simulink model "MotorDC_Simscape"  (R2026a)
settings: Solver=ode23t  StopTime=5
values from neighbouring files (symbols this model uses):
  b = 0.0012    [crear_motor_simscape.m]    (also in crear_motor_simulink.m; mat.m)
  Kt = 0.01    [crear_motor_simscape.m]    (also in crear_motor_simulink.m; mat.m)
  Ra = 2    [crear_motor_simscape.m]    (also in crear_motor_simulink.m; mat.m)
libraries: fl_lib x10, nesl_utility x4
settings Model: Creator=jmlc2  LastModifiedBy=jmlc2

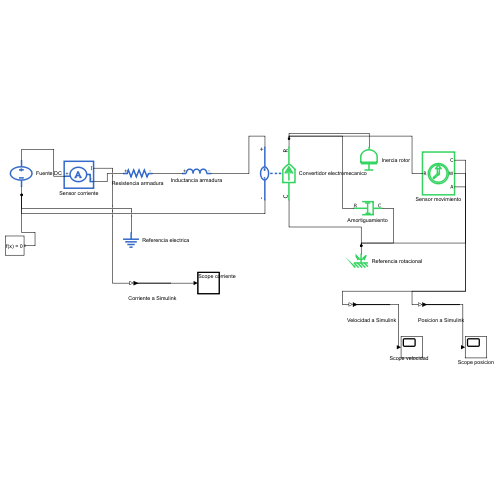
[thumbnail: Simulink's stored preview of the top-level diagram]
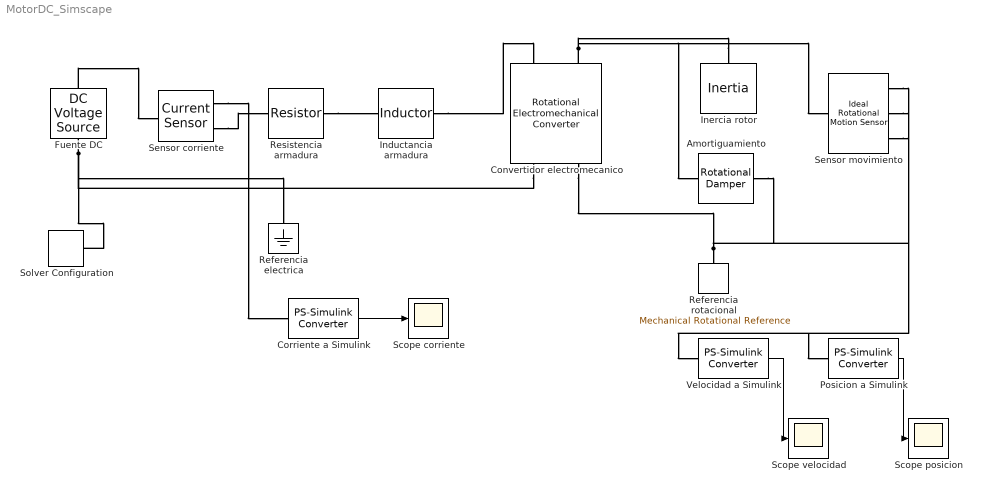
== system MotorDC_Simscape ==
  Amortiguamiento : fl_lib/Mechanical/Rotational Elements/Rotational Damper  D=b N*m*s/rad  w_specify=off  w_priority=None  w=0 rad/s  w_nominal_specify=off  w_nominal_value=1  w_nominal_unit=rad/s  t_specify=off  t_priority=None  t=0 N*m  t_nominal_specify=off  t_nominal_value=1  t_nominal_unit=N*m
  Convertidor electromecanico : fl_lib/Electrical/Electrical Elements/Rotational Electromechanical Converter  K=Kt V*s/rad  i_specify=off  i_priority=None  i=0 A  i_nominal_specify=off  i_nominal_value=1  i_nominal_unit=A  v_specify=off  v_priority=None  v=0 V  v_nominal_specify=off  v_nominal_value=1  v_nominal_unit=V  t_specify=off  t_priority=None  t=0 N*m  t_nominal_specify=off  t_nominal_value=1  t_nominal_unit=N*m  w_specify=off  w_priority=None  w=0 rad/s  w_nominal_specify=off  w_nominal_value=1  w_nominal_unit=rad/s
  Corriente a Simulink : nesl_utility/PS-Simulink Converter  PhysicalDomain=network_engine_domain  SubClassName=ps_output  LeftPortType=input  RightPortType=output  PseudoPeriodic=off  Frequencies=[]  VectorFormat=inherit  Unit=A  AffineConversion=off
  Fuente DC : fl_lib/Electrical/Electrical Sources/DC Voltage Source  v0=va V
  Inductancia armadura : fl_lib/Electrical/Electrical Elements/Inductor  l=La H  r=0 Ohm  g=1e-9 1/Ohm  i_specify=off  i_priority=None  i=0 A  i_nominal_specify=off  i_nominal_value=1  i_nominal_unit=A  v_specify=off  v_priority=None  v=0 V  v_nominal_specify=off  v_nominal_value=1  v_nominal_unit=V  i_L_specify=off  i_L_priority=High  i_L=0 A  i_L_nominal_specify=off  i_L_nominal_value=1  i_L_nominal_unit=A
  Inercia rotor : fl_lib/Mechanical/Rotational Elements/Inertia  inertia=J kg*m^2  num_ports=foundation.enum.numPorts2.one  w_specify=off  w_priority=High  w=0 rad/s  w_nominal_specify=off  w_nominal_value=1  w_nominal_unit=rad/s  t_specify=off  t_priority=None  t=0 N*m  t_nominal_specify=off  t_nominal_value=1  t_nominal_unit=N*m
  Posicion a Simulink : nesl_utility/PS-Simulink Converter  PhysicalDomain=network_engine_domain  SubClassName=ps_output  LeftPortType=input  RightPortType=output  PseudoPeriodic=off  Frequencies=[]  VectorFormat=inherit  Unit=rad  AffineConversion=off
  Referencia electrica : fl_lib/Electrical/Electrical Elements/Electrical Reference
  Referencia rotacional : fl_lib/Mechanical/Rotational Elements/Mechanical Rotational Reference
  Resistencia armadura : fl_lib/Electrical/Electrical Elements/Resistor  R=Ra Ohm  i_specify=off  i_priority=None  i=0 A  i_nominal_specify=off  i_nominal_value=1  i_nominal_unit=A  v_specify=off  v_priority=None  v=0 V  v_nominal_specify=off  v_nominal_value=1  v_nominal_unit=V
  Scope corriente : Scope
      settings: TimeSpan=5  ActiveDisplayYMinimum=0  ActiveDisplayYMaximum=6
  Scope posicion : Scope
      settings: TimeSpan=5  ActiveDisplayYMinimum=0  ActiveDisplayYMaximum=250
  Scope velocidad : Scope
      settings: TimeSpan=5  ActiveDisplayYMinimum=0  ActiveDisplayYMaximum=50
  Sensor corriente : fl_lib/Electrical/Electrical Sensors/Current Sensor
  Sensor movimiento : fl_lib/Mechanical/Mechanical Sensors/Ideal Rotational Motion Sensor  reference=foundation.enum.MeasurementReference.difference  acceleration_port=false  velocity_port=true  position_port=true  wrap_angle=false  offset=0 rad
  Solver Configuration : nesl_utility/Solver Configuration  PhysicalDomain=network_engine_domain  SubClassName=solver  LeftPortType=input  RightPortType=generic  Tones=[]  Harmonics=[]  SimulateNoise=off  Profile=off  UseLocalSampling=off  EnableSwitchedLinearOptims=on  FrequencyDomain=off  UseCCode=off  RelTol=0.001  AbsTol=0.001  MinStep=1e-09  ToWorkspace=off  RevertToSquareIcSolve=off  NumHomotopyIterations=100  PhasorMode=off  PhasorModeNumHarmonics=1  ConsistencySolver=NEWTON_XTOL_AFTER_FTOL  CanonicalOrdering=CANONICAL  OptimizeIntermediates=OPTIMIZED  IndexReductionMethod=DerivativeReplacement  DoDC=off  ResidualTolerance=1e-09  ConsistencyTolSource=GLOBAL  ConsistencyAbsTol=0.001  ConsistencyRelTol=0.001  ConsistencyTolFactor=0.001  UseLocalSolver=off  LocalSolverChoice=NE_BACKWARD_EULER_ADVANCER  ResolveIndetEquations=on  FunctionEvalNumThread=1  LocalSolverSampleTime=0.001  DoFixedCost=off  MaxNonlinIter=3  MaxModeIter=2  ComputeImpulses=off  ImpulseIterations=2  LinearAlgebra=auto  LinearAlgebraNumThread=0  EquationFormulation=NE_TIME_EF  DelaysMemoryBudget=1024  AutomaticFiltering=on  FilteringTimeConstant=0.001  PartitionStorageMethod=AS_NEEDED  PartitionMemoryBudget=1024  PartitionMethod=ROBUST  MultibodyUseLocalSolver=off  MultibodyLocalSolverChoice=ODE1  MultibodyLocalSolverSampleTime=0.001
  Velocidad a Simulink : nesl_utility/PS-Simulink Converter  PhysicalDomain=network_engine_domain  SubClassName=ps_output  LeftPortType=input  RightPortType=output  PseudoPeriodic=off  Frequencies=[]  VectorFormat=inherit  Unit=rad/s  AffineConversion=off
  wires:
  Corriente a Simulink/1 -> Scope corriente/1
  Velocidad a Simulink/1 -> Scope velocidad/1
  Posicion a Simulink/1 -> Scope posicion/1
  connections:
  Fuente DC/LConn1 -- Sensor corriente/LConn1
  Sensor corriente/RConn2 -- Resistencia armadura/LConn1
  Resistencia armadura/RConn1 -- Inductancia armadura/LConn1
  Inductancia armadura/RConn1 -- Convertidor electromecanico/LConn1
  Convertidor electromecanico/RConn1 -- Referencia electrica/LConn1 -- Fuente DC/RConn1 -- Solver Configuration/RConn1
  Inercia rotor/LConn1 -- Convertidor electromecanico/LConn2 -- Amortiguamiento/LConn1 -- Sensor movimiento/LConn1
  Amortiguamiento/RConn1 -- Convertidor electromecanico/RConn2 -- Referencia rotacional/LConn1 -- Sensor movimiento/RConn1
  Sensor corriente/RConn1 -- Corriente a Simulink/LConn1
  Sensor movimiento/RConn2 -- Velocidad a Simulink/LConn1
  Sensor movimiento/RConn3 -- Posicion a Simulink/LConn1
